simulink model "mars_rover_test_harness_chassis"  (R2025a)
settings: Solver=ode23t  StartTime=0.0  StopTime=30  FixedStep=1e-10  MaxStep=1e-1  RelTol=1e-3  AbsTol=1e-3  EnableMultiTasking=on
undefined symbols (not defined in the file): arm_q0, Control, L1, L2, L3, LS1, LS3, R1, R2, R3, Rover, RS1, RS3, X, Y, Z
libraries: sm_lib x119, nesl_utility x99, fl_lib x85, sdl_lib x20, ee_lib x10, mars_rover_lib x8, simulink x5, slpidlib x3, batteryecm_lib x2
(part 4 of 8)

== system mars_rover_test_harness_chassis/Rover/Chassis/Camera/rsm_base_1_RIGID ==
  ReferenceFrame : sm_lib/Frames and Transforms/Reference Frame
  Solid : sm_lib/Body Elements/File Solid  ExtGeomFileName=rover_chassis_sensor_base.stl  UnitType=Custom  ExtGeomFileUnits=cm  StepReaderType=HEX  ExportConvexHullGeometry=off  InertiaType=CalculateFromGeometry  BasedOnType=Density  Density=2000  DensityUnits=kg/m^3  Mass=202690.508551217  MassUnits=kg  CenterOfMass=[-2.09994238818055e-07 21.8231915316941 -2.20167989735098e-07]  CenterOfMassUnits=m  MomentsOfInertia=[2411866.97125594 5940029.20050206 6701187.74240286]  MomentsOfInertiaUnits=kg*m^2  ProductsOfInertia=[0.00792234309140369 -0.0164088810985133 -0.460936358460458]  ProductsOfInertiaUnits=kg*m^2  GraphicType=FromGeometry  MarkerShape=Sphere  MarkerSize=10  GraphicVisPropType=SimpleVisualProperties  GraphicDiffuseColor=[0.2 0.2 0.2]  GraphicOpacity=1  GraphicSpecularColor=[0.5 0.5 0.5 1.0]  GraphicAmbientColor=[0.15 0.15 0.15 1.0]  GraphicEmissiveColor=[0.0 0.0 0.0 1.0]  GraphicShininess=75  DoExposeReferenceFrame=on  SerializedFrames=<Frames/>
  Transform : sm_lib/Frames and Transforms/Rigid Transform  RotationMethod=ArbitraryAxis  FollAlignAxisA=+X  BaseAlignAxisA=+Y  FollAlignAxisB=+Y  BaseAlignAxisB=+Z  RotationStandardAxis=+Z  RotationAngle=2.0943951023932  RotationAngleUnits=rad  RotationArbitraryAxis=[0.577350269189626 0.577350269189626 0.577350269189626]  RotationSequenceAxes=FollowerAxes  RotationSequence=XYX  RotationSequenceAngles=[0 0 0]  RotationSequenceAnglesUnits=deg  RotationMatrix=[1 0 0; 0 1 0; 0 0 1]  Quaternion=[1 0 0 0]  TranslationMethod=Cartesian  TranslationCartesianOffset=[-40 220.000003786473 -2.05636384635e-06]  TranslationCartesianOffsetUnits=mm  TranslationStandardAxis=+Z  TranslationStandardOffset=0  TranslationStandardOffsetUnits=mm  TranslationROffset=0  TranslationROffsetUnits=m  TranslationThetaOffset=0  TranslationThetaOffsetUnits=deg  TranslationZOffset=0  TranslationZOffsetUnits=m
  F : PMIOPort  Side=Right
  F1 : PMIOPort  Port=2  Side=Left
  connections:
  Transform/LConn1 -- F1/RConn1 -- ReferenceFrame/RConn1 -- Solid/RConn1
  Transform/RConn1 -- F/RConn1

== system mars_rover_test_harness_chassis/Rover/Chassis/Camera/rsm_head_1_RIGID ==
  Reference Camera : sm_lib/Frames and Transforms/Reference Frame
  ReferenceFrame : sm_lib/Frames and Transforms/Reference Frame
  Rigid Transform : sm_lib/Frames and Transforms/Rigid Transform  RotationMethod=StandardAxis  FollAlignAxisA=+X  BaseAlignAxisA=+Y  FollAlignAxisB=+Y  BaseAlignAxisB=+Z  RotationStandardAxis=+X  RotationAngle=-90  RotationAngleUnits=deg  RotationArbitraryAxis=[0 0 1]  RotationSequenceAxes=FollowerAxes  RotationSequence=XYX  RotationSequenceAngles=[0 0 0]  RotationSequenceAnglesUnits=deg  RotationMatrix=[1 0 0; 0 1 0; 0 0 1]  Quaternion=[1 0 0 0]  TranslationMethod=Cartesian  TranslationCartesianOffset=[12 11 13]  TranslationCartesianOffsetUnits=cm  TranslationStandardAxis=+Z  TranslationStandardOffset=0  TranslationStandardOffsetUnits=cm  TranslationROffset=0  TranslationROffsetUnits=m  TranslationThetaOffset=0  TranslationThetaOffsetUnits=deg  TranslationZOffset=0  TranslationZOffsetUnits=m
  Solid : sm_lib/Body Elements/File Solid  ExtGeomFileName=rover_chassis_sensor_head.stl  UnitType=Custom  ExtGeomFileUnits=cm  StepReaderType=HEX  ExportConvexHullGeometry=off  InertiaType=CalculateFromGeometry  BasedOnType=Density  Density=2000  DensityUnits=kg/m^3  Mass=1  MassUnits=kg  CenterOfMass=[-0.00288550161429388 71.0000014663329 -4.54954138701768e-07]  CenterOfMassUnits=m  MomentsOfInertia=[1608495.92335293 6519098.97331966 6519098.97331985]  MomentsOfInertiaUnits=kg*m^2  ProductsOfInertia=[-6.49609544482223e-08 0.336731288221059 1.08955853960892]  ProductsOfInertiaUnits=kg*m^2  GraphicType=FromGeometry  MarkerShape=Sphere  MarkerSize=10  GraphicVisPropType=SimpleVisualProperties  GraphicDiffuseColor=[0.8 0.5 0.3]  GraphicOpacity=1  GraphicSpecularColor=[1 1 1 1.0]  GraphicAmbientColor=[0.15 0.15 0.15 0.8]  GraphicEmissiveColor=[0 0 0 1]  GraphicShininess=90  DoExposeReferenceFrame=on  SerializedFrames=<Frames/>
  Transform : sm_lib/Frames and Transforms/Rigid Transform  RotationMethod=ArbitraryAxis  FollAlignAxisA=+X  BaseAlignAxisA=+Y  FollAlignAxisB=+Y  BaseAlignAxisB=+Z  RotationStandardAxis=+Z  RotationAngle=2.0943951023932  RotationAngleUnits=rad  RotationArbitraryAxis=[0.577350269189626 0.577350269189626 0.577350269189626]  RotationSequenceAxes=FollowerAxes  RotationSequence=XYX  RotationSequenceAngles=[0 0 0]  RotationSequenceAnglesUnits=deg  RotationMatrix=[1 0 0; 0 1 0; 0 0 1]  Quaternion=[1 0 0 0]  TranslationMethod=Cartesian  TranslationCartesianOffset=[-40.5288600921631 710.000004438766 -7.70947271803379e-06]  TranslationCartesianOffsetUnits=mm  TranslationStandardAxis=+Z  TranslationStandardOffset=0  TranslationStandardOffsetUnits=mm  TranslationROffset=0  TranslationROffsetUnits=m  TranslationThetaOffset=0  TranslationThetaOffsetUnits=deg  TranslationZOffset=0  TranslationZOffsetUnits=m
  F : PMIOPort  Side=Left
  connections:
  ReferenceFrame/RConn1 -- Solid/RConn1 -- Transform/LConn1
  Transform/RConn1 -- F/RConn1 -- Rigid Transform/LConn1
  Rigid Transform/RConn1 -- Reference Camera/RConn1

== system mars_rover_test_harness_chassis/Rover/Chassis/Camera/rsm_lower_mast_2_RIGID ==
  ReferenceFrame : sm_lib/Frames and Transforms/Reference Frame
  Solid : sm_lib/Body Elements/File Solid  ExtGeomFileName=rover_chassis_sensor_mast_lower.stl  UnitType=Custom  ExtGeomFileUnits=cm  StepReaderType=HEX  ExportConvexHullGeometry=off  InertiaType=CalculateFromGeometry  BasedOnType=Density  Density=2000  DensityUnits=kg/m^3  Mass=403410.668072862  MassUnits=kg  CenterOfMass=[4.00000000041938 10.1119460218271 35.0000011171366]  CenterOfMassUnits=m  MomentsOfInertia=[4810006.95412572 3779509.77447628 5346172.06825756]  MomentsOfInertiaUnits=kg*m^2  ProductsOfInertia=[0.0256104910578052 9.59441184474277e-11 -0.00591852250388119]  ProductsOfInertiaUnits=kg*m^2  GraphicType=FromGeometry  MarkerShape=Sphere  MarkerSize=10  GraphicVisPropType=SimpleVisualProperties  GraphicDiffuseColor=[1 1 0.8]  GraphicOpacity=1  GraphicSpecularColor=[0.5 0.5 0.5 1.0]  GraphicAmbientColor=[0.15 0.15 0.15 1.0]  GraphicEmissiveColor=[0.0 0.0 0.0 1.0]  GraphicShininess=75  DoExposeReferenceFrame=on  SerializedFrames=<Frames/>
  Transform : sm_lib/Frames and Transforms/Rigid Transform  RotationMethod=ArbitraryAxis  FollAlignAxisA=+X  BaseAlignAxisA=+Y  FollAlignAxisB=+Y  BaseAlignAxisB=+Z  RotationStandardAxis=+Z  RotationAngle=2.0943951023932  RotationAngleUnits=rad  RotationArbitraryAxis=[-0.577350269189626 -0.577350269189626 -0.577350269189626]  RotationSequenceAxes=FollowerAxes  RotationSequence=XYX  RotationSequenceAngles=[0 0 0]  RotationSequenceAnglesUnits=deg  RotationMatrix=[1 0 0; 0 1 0; 0 0 1]  Quaternion=[1 0 0 0]  TranslationMethod=Cartesian  TranslationCartesianOffset=[40.0000013147577 450.900022888183 350.000005500325]  TranslationCartesianOffsetUnits=mm  TranslationStandardAxis=+Z  TranslationStandardOffset=0  TranslationStandardOffsetUnits=mm  TranslationROffset=0  TranslationROffsetUnits=m  TranslationThetaOffset=0  TranslationThetaOffsetUnits=deg  TranslationZOffset=0  TranslationZOffsetUnits=m
  Transform1 : sm_lib/Frames and Transforms/Rigid Transform  RotationMethod=ArbitraryAxis  FollAlignAxisA=+X  BaseAlignAxisA=+Y  FollAlignAxisB=+Y  BaseAlignAxisB=+Z  RotationStandardAxis=+Z  RotationAngle=2.0943951023932  RotationAngleUnits=rad  RotationArbitraryAxis=[0.577350269189626 0.577350269189626 0.577350269189626]  RotationSequenceAxes=FollowerAxes  RotationSequence=XYX  RotationSequenceAngles=[0 0 0]  RotationSequenceAnglesUnits=deg  RotationMatrix=[1 0 0; 0 1 0; 0 0 1]  Quaternion=[1 0 0 0]  TranslationMethod=Cartesian  TranslationCartesianOffset=[0 100.000002423247 350.000011189513]  TranslationCartesianOffsetUnits=mm  TranslationStandardAxis=+Z  TranslationStandardOffset=0  TranslationStandardOffsetUnits=mm  TranslationROffset=0  TranslationROffsetUnits=m  TranslationThetaOffset=0  TranslationThetaOffsetUnits=deg  TranslationZOffset=0  TranslationZOffsetUnits=m
  F1 : PMIOPort  Side=Left
  F : PMIOPort  Port=2  Side=Right
  connections:
  Transform/LConn1 -- Transform1/LConn1 -- ReferenceFrame/RConn1 -- Solid/RConn1
  Transform/RConn1 -- F/RConn1
  Transform1/RConn1 -- F1/RConn1

== system mars_rover_test_harness_chassis/Rover/Chassis/Camera/rsm_outer_ring_1_RIGID ==
  ReferenceFrame : sm_lib/Frames and Transforms/Reference Frame
  Rigid Transform : sm_lib/Frames and Transforms/Rigid Transform  RotationMethod=StandardAxis  FollAlignAxisA=+X  BaseAlignAxisA=+Y  FollAlignAxisB=+Y  BaseAlignAxisB=+Z  RotationStandardAxis=+Z  RotationAngle=20.0  RotationAngleUnits=deg  RotationArbitraryAxis=[0 0 1]  RotationSequenceAxes=FollowerAxes  RotationSequence=XYX  RotationSequenceAngles=[0 0 0]  RotationSequenceAnglesUnits=deg  RotationMatrix=[1 0 0; 0 1 0; 0 0 1]  Quaternion=[1 0 0 0]  TranslationMethod=None  TranslationCartesianOffset=[0 0 0]  TranslationCartesianOffsetUnits=m  TranslationStandardAxis=+Z  TranslationStandardOffset=0  TranslationStandardOffsetUnits=m  TranslationROffset=0  TranslationROffsetUnits=m  TranslationThetaOffset=0  TranslationThetaOffsetUnits=deg  TranslationZOffset=0  TranslationZOffsetUnits=m
  Solid : sm_lib/Body Elements/File Solid  ExtGeomFileName=rover_chassis_sensor_ring_outer.stl  UnitType=Custom  ExtGeomFileUnits=cm  StepReaderType=HEX  ExportConvexHullGeometry=off  InertiaType=CalculateFromGeometry  BasedOnType=Density  Density=2000  DensityUnits=kg/m^3  Mass=2000  MassUnits=kg  CenterOfMass=[3.99999986837507 43.0793255522792 35.0000003648552]  CenterOfMassUnits=m  MomentsOfInertia=[35996.0863503472 57529.9697773705 35996.0863503472]  MomentsOfInertiaUnits=kg*m^2  ProductsOfInertia=[0.000493832044278217 -4.64395705120422e-11 0.00068000513182705]  ProductsOfInertiaUnits=kg*m^2  GraphicType=FromGeometry  MarkerShape=Sphere  MarkerSize=10  GraphicVisPropType=SimpleVisualProperties  GraphicDiffuseColor=[0.2 0.2 0.2]  GraphicOpacity=1  GraphicSpecularColor=[0.5 0.5 0.5 1.0]  GraphicAmbientColor=[0.15 0.15 0.15 1.0]  GraphicEmissiveColor=[0.0 0.0 0.0 1.0]  GraphicShininess=75  DoExposeReferenceFrame=on  SerializedFrames=<Frames/>
  Transform : sm_lib/Frames and Transforms/Rigid Transform  RotationMethod=ArbitraryAxis  FollAlignAxisA=+X  BaseAlignAxisA=+Y  FollAlignAxisB=+Y  BaseAlignAxisB=+Z  RotationStandardAxis=+Z  RotationAngle=2.09439510239319  RotationAngleUnits=rad  RotationArbitraryAxis=[-0.577350269189626 -0.577350269189627 -0.577350269189625]  RotationSequenceAxes=FollowerAxes  RotationSequence=XYX  RotationSequenceAngles=[0 0 0]  RotationSequenceAnglesUnits=deg  RotationMatrix=[1 0 0; 0 1 0; 0 0 1]  Quaternion=[1 0 0 0]  TranslationMethod=Cartesian  TranslationCartesianOffset=[39.9999957537947 420.900022888184 350.000001520764]  TranslationCartesianOffsetUnits=mm  TranslationStandardAxis=+Z  TranslationStandardOffset=0  TranslationStandardOffsetUnits=mm  TranslationROffset=0  TranslationROffsetUnits=m  TranslationThetaOffset=0  TranslationThetaOffsetUnits=deg  TranslationZOffset=0  TranslationZOffsetUnits=m
  Transform1 : sm_lib/Frames and Transforms/Rigid Transform  RotationMethod=ArbitraryAxis  FollAlignAxisA=+X  BaseAlignAxisA=+Y  FollAlignAxisB=+Y  BaseAlignAxisB=+Z  RotationStandardAxis=+Z  RotationAngle=2.29441736937637  RotationAngleUnits=rad  RotationArbitraryAxis=[-0.450882585021863 -0.631151683244211 -0.631151683244211]  RotationSequenceAxes=FollowerAxes  RotationSequence=XYX  RotationSequenceAngles=[0 0 0]  RotationSequenceAnglesUnits=deg  RotationMatrix=[1 0 0; 0 1 0; 0 0 1]  Quaternion=[1 0 0 0]  TranslationMethod=Cartesian  TranslationCartesianOffset=[39.9999957537972 461.900007629394 350.000001520762]  TranslationCartesianOffsetUnits=mm  TranslationStandardAxis=+Z  TranslationStandardOffset=0  TranslationStandardOffsetUnits=mm  TranslationROffset=0  TranslationROffsetUnits=m  TranslationThetaOffset=0  TranslationThetaOffsetUnits=deg  TranslationZOffset=0  TranslationZOffsetUnits=m
  F1 : PMIOPort  Side=Left
  F : PMIOPort  Port=2  Side=Left
  connections:
  Transform/LConn1 -- Transform1/LConn1 -- ReferenceFrame/RConn1 -- Solid/RConn1
  Transform/RConn1 -- F/RConn1
  Rigid Transform/RConn1 -- F1/RConn1
  Rigid Transform/LConn1 -- Transform1/RConn1

== system mars_rover_test_harness_chassis/Rover/Chassis/Camera/rsm_upper_mast_1_RIGID ==
  ReferenceFrame : sm_lib/Frames and Transforms/Reference Frame
  Solid : sm_lib/Body Elements/File Solid  ExtGeomFileName=rover_chassis_sensor_mast_upper.stl  UnitType=Custom  ExtGeomFileUnits=cm  StepReaderType=HEX  ExportConvexHullGeometry=off  InertiaType=CalculateFromGeometry  BasedOnType=Density  Density=2000  DensityUnits=kg/m^3  Mass=382776.497765057  MassUnits=kg  CenterOfMass=[3.99998590581562 58.9787952931336 34.9999786232352]  CenterOfMassUnits=m  MomentsOfInertia=[3038949.11550358 3496444.12832479 3624138.33109519]  MomentsOfInertiaUnits=kg*m^2  ProductsOfInertia=[-149.383305940768 -0.0992863146641867 -86.2313374210248]  ProductsOfInertiaUnits=kg*m^2  GraphicType=FromGeometry  MarkerShape=Sphere  MarkerSize=10  GraphicVisPropType=SimpleVisualProperties  GraphicDiffuseColor=[1 1 0.8]  GraphicOpacity=1  GraphicSpecularColor=[0.5 0.5 0.5 1.0]  GraphicAmbientColor=[0.15 0.15 0.15 1.0]  GraphicEmissiveColor=[0.0 0.0 0.0 1.0]  GraphicShininess=75  DoExposeReferenceFrame=on  SerializedFrames=<Frames/>
  Transform : sm_lib/Frames and Transforms/Rigid Transform  RotationMethod=ArbitraryAxis  FollAlignAxisA=+X  BaseAlignAxisA=+Y  FollAlignAxisB=+Y  BaseAlignAxisB=+Z  RotationStandardAxis=+Z  RotationAngle=2.0943951023932  RotationAngleUnits=rad  RotationArbitraryAxis=[-0.577350269189626 -0.577350269189626 -0.577350269189626]  RotationSequenceAxes=FollowerAxes  RotationSequence=XYX  RotationSequenceAngles=[0 0 0]  RotationSequenceAnglesUnits=deg  RotationMatrix=[1 0 0; 0 1 0; 0 0 1]  Quaternion=[1 0 0 0]  TranslationMethod=Cartesian  TranslationCartesianOffset=[39.8936241533249 429.9 349.815749642353]  TranslationCartesianOffsetUnits=mm  TranslationStandardAxis=+Z  TranslationStandardOffset=0  TranslationStandardOffsetUnits=mm  TranslationROffset=0  TranslationROffsetUnits=m  TranslationThetaOffset=0  TranslationThetaOffsetUnits=deg  TranslationZOffset=0  TranslationZOffsetUnits=m
  Transform1 : sm_lib/Frames and Transforms/Rigid Transform  RotationMethod=ArbitraryAxis  FollAlignAxisA=+X  BaseAlignAxisA=+Y  FollAlignAxisB=+Y  BaseAlignAxisB=+Z  RotationStandardAxis=+Z  RotationAngle=2.0943951023932  RotationAngleUnits=rad  RotationArbitraryAxis=[0.577350269189626 0.577350269189626 0.577350269189626]  RotationSequenceAxes=FollowerAxes  RotationSequence=XYX  RotationSequenceAngles=[0 0 0]  RotationSequenceAnglesUnits=deg  RotationMatrix=[1 0 0; 0 1 0; 0 0 1]  Quaternion=[1 0 0 0]  TranslationMethod=Cartesian  TranslationCartesianOffset=[7.105427357601e-14 590.000009936775 350.000030393688]  TranslationCartesianOffsetUnits=mm  TranslationStandardAxis=+Z  TranslationStandardOffset=0  TranslationStandardOffsetUnits=mm  TranslationROffset=0  TranslationROffsetUnits=m  TranslationThetaOffset=0  TranslationThetaOffsetUnits=deg  TranslationZOffset=0  TranslationZOffsetUnits=m
  F : PMIOPort  Side=Left
  F1 : PMIOPort  Port=2  Side=Right
  connections:
  Transform/LConn1 -- Transform1/LConn1 -- ReferenceFrame/RConn1 -- Solid/RConn1
  Transform/RConn1 -- F/RConn1
  Transform1/RConn1 -- F1/RConn1

== system mars_rover_test_harness_chassis/Rover/Chassis/Powertrain/Electrical ==
  In Bus Element : Inport  PortName=Trq  Element=Steer
  In Bus Element1 : Inport  PortName=Trq  Element=Drive
  Drive : Subsystem  mask{trq_max=Rover.Powertrain.Drive.Motor.max_torque, power_max=Rover.Powertrain.Drive.Motor.max_power, trq_tc=Rover.Powertrain.Drive.Motor.tc_torque, eff_overall=Rover.Powertrain.Drive.Motor.efficiency, eff_spd=Rover.Powertrain.Drive.Motor.eff_meas_spd, eff_trq=Rover.Powertrain.Drive.Motor.eff_meas_trq, rotor_d=Rover.Powertrain.Drive.Motor.damping, drive_ratio=Rover.Powertrain.Drive.Motor.gear_ratio}
      mask prompts: trq_max "Max Torque (N*m)"; power_max "Max Power (W)"; trq_tc "Time Constant, Torque (s)"; eff_overall "Efficiency (%)"; eff_spd "Speed for Efficiency (rpm)"; eff_trq "Torque for Efficiency (N*m)"; rotor_d "Rotor Damping (N*m/(rad/s))"; drive_ratio "Drive Ratio"
      mask Display: image('mars_rover_terrain_motor_elec_drive.png');
  Mechanical Rotational Reference : fl_lib/Mechanical/Rotational Elements/Mechanical Rotational Reference
  Power : Subsystem
      mask Display: image('mars_rover_terrain_battery.png');
  Steer : Subsystem  mask{trq_max=Rover.Powertrain.Steer.Motor.max_torque, power_max=Rover.Powertrain.Steer.Motor.max_power, trq_tc=Rover.Powertrain.Steer.Motor.tc_torque, eff_overall=Rover.Powertrain.Steer.Motor.efficiency, eff_spd=Rover.Powertrain.Steer.Motor.eff_meas_spd, eff_trq=Rover.Powertrain.Steer.Motor.eff_meas_trq, rotor_d=Rover.Powertrain.Steer.Motor.damping, drive_ratio=Rover.Powertrain.Steer.Motor.gear_ratio}
      mask prompts: trq_max "Max Torque (N*m)"; power_max "Max Power (W)"; trq_tc "Time Constant, Torque (s)"; eff_overall "Efficiency (%)"; eff_spd "Speed for Efficiency (rpm)"; eff_trq "Torque for Efficiency (N*m)"; rotor_d "Rotor Damping (N*m/(rad/s))"; drive_ratio "Drive Ratio"
      mask Display: image('mars_rover_terrain_motor_elec_steer.png');
  S : PMIOPort  Side=Right
  Out Bus Element : Outport  PortName=m  Element=Drive
  Out Bus Element1 : Outport  PortName=m  Element=Steer
  Out Bus Element2 : Outport  PortName=m  Element=Battery
  wires:
  In Bus Element/1 -> Steer/1(Trq)
  In Bus Element1/1 -> Drive/1(Trq)
  Steer/1(m) -> Out Bus Element1/1
  Drive/1(m) -> Out Bus Element/1
  Power/1(m) -> Out Bus Element2/1
  connections:
  S/RConn1 -- Drive/RConn1 -- Steer/RConn1
  Power/RConn1 -- Drive/LConn1 -- Steer/LConn1
  Mechanical Rotational Reference/LConn1 -- Drive/RConn2 -- Steer/RConn2
  Power/RConn2 -- Drive/LConn2 -- Steer/LConn2

== system mars_rover_test_harness_chassis/Rover/Chassis/Powertrain/Ideal ==
  In Bus Element6 : Inport  PortName=Trq  Element=Steer
  In Bus Element : Inport  PortName=Trq  Element=Drive
  Calculate Power : Subsystem
  Drive : Subsystem  mask{drive_ratio=Rover.Powertrain.Drive.Motor.gear_ratio, motor_d=Rover.Powertrain.Drive.Motor.damping, motor_tc=Rover.Powertrain.Drive.Motor.tc_torque}
      mask prompts: drive_ratio "Drive Ratio"; motor_d "Motor Damping (N*m/(rad/s))"; motor_tc "Motor Time Constant"
      mask Display: image('mars_rover_terrain_motor_ideal_drive.png');
  Mechanical Rotational Reference : fl_lib/Mechanical/Rotational Elements/Mechanical Rotational Reference
  Power : Subsystem
      mask Display: image('mars_rover_terrain_battery.png');
  Steer : Subsystem  mask{drive_ratio=Rover.Powertrain.Drive.Motor.gear_ratio, motor_d=Rover.Powertrain.Steer.Motor.damping, motor_tc=Rover.Powertrain.Steer.Motor.tc_torque}
      mask prompts: drive_ratio "Gear Ratio"; motor_d "Motor Damping (N*m/(rad/s))"; motor_tc "Motor Time Constant"
      mask Display: image('mars_rover_terrain_motor_ideal_steer.png')
  S : PMIOPort  Side=Right
  Out Bus Element : Outport  PortName=m  Element=Steer
  Out Bus Element1 : Outport  PortName=m  Element=Drive
  Out Bus Element2 : Outport  PortName=m  Element=Battery
  wires:
  Steer/1(m) -> Out Bus Element/1, [S]
  In Bus Element6/1 -> Steer/1(Trq)
  Drive/1(m) -> [D], Out Bus Element1/1
  In Bus Element/1 -> Drive/1(Trq)
  [S] -> Calculate Power/1(S)
  [D] -> Calculate Power/2(D)
  Calculate Power/1(i) -> Power/1(i)
  Power/1(m) -> Out Bus Element2/1
  connections:
  Steer/RConn1 -- Drive/RConn1 -- S/RConn1
  Mechanical Rotational Reference/LConn1 -- Steer/LConn1 -- Drive/LConn1

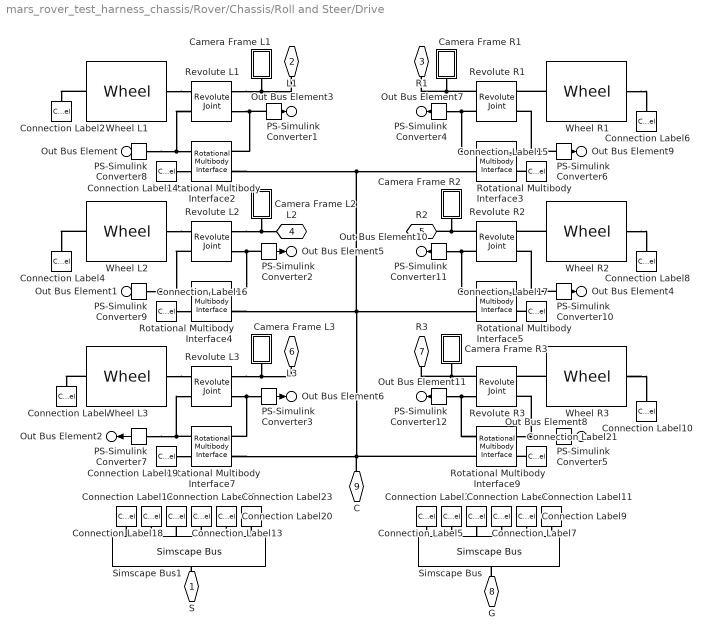
== system mars_rover_test_harness_chassis/Rover/Chassis/Roll and Steer/Drive ==
  Camera Frame L1 : Subsystem
  Camera Frame L2 : Subsystem
  Camera Frame L3 : Subsystem
  Camera Frame R1 : Subsystem
  Camera Frame R2 : Subsystem
  Camera Frame R3 : Subsystem
  Connection Label : ConnectionLabel  Label=GL3
  Connection Label1 : ConnectionLabel  Label=GL3
  Connection Label10 : ConnectionLabel  Label=GR3
  Connection Label11 : ConnectionLabel  Label=GR3
  Connection Label12 : ConnectionLabel  Label=L1
  Connection Label13 : ConnectionLabel  Label=R1
  Connection Label14 : ConnectionLabel  Label=L1
  Connection Label15 : ConnectionLabel  Label=R1
  Connection Label16 : ConnectionLabel  Label=L2
  Connection Label17 : ConnectionLabel  Label=R2
  Connection Label18 : ConnectionLabel  Label=L2
  Connection Label19 : ConnectionLabel  Label=L3
  Connection Label2 : ConnectionLabel  Label=GL1
  Connection Label20 : ConnectionLabel  Label=R2
  Connection Label21 : ConnectionLabel  Label=R3
  Connection Label22 : ConnectionLabel  Label=L3
  Connection Label23 : ConnectionLabel  Label=R3
  Connection Label3 : ConnectionLabel  Label=GL1
  Connection Label4 : ConnectionLabel  Label=GL2
  Connection Label5 : ConnectionLabel  Label=GL2
  Connection Label6 : ConnectionLabel  Label=GR1
  Connection Label7 : ConnectionLabel  Label=GR1
  Connection Label8 : ConnectionLabel  Label=GR2
  Connection Label9 : ConnectionLabel  Label=GR2
  PS-Simulink Converter{1..12} (12 alike) : nesl_utility/PS-Simulink Converter  PhysicalDomain=network_engine_domain  SubClassName=ps_output  LeftPortType=input  RightPortType=output  PseudoPeriodic=off  Frequencies=[]  VectorFormat=1-D array  Unit=inherit  AffineConversion=off
  Revolute L1 : sm_lib/Joints/Revolute Joint  JointMode=Normal  CompositeWrenchDir=FollowerOnBase  CompositeWrenchFrame=BaseFrame  SenseConstraintForce=off  SenseConstraintTorque=off  SenseTotalForce=off  SenseTotalTorque=off  PositionTargetSpecify=off  PositionTargetPriority=High  PositionTargetValue=0  PositionTargetValueUnits=deg  VelocityTargetSpecify=off  VelocityTargetPriority=High  VelocityTargetValue=0  VelocityTargetValueUnits=deg/s  EquilibriumPosition=0  EquilibriumPositionUnits=deg  SpringStiffness=0  SpringStiffnessUnits=N*m/deg  DampingCoefficient=Rover.Drive.D  DampingCoefficientUnits=N*m/(deg/s)  LowerLimitSpecify=off  LowerLimitBound=-90  LowerLimitBoundUnits=deg  LowerLimitStiffness=1e4  LowerLimitStiffnessUnits=N*m/deg  LowerLimitDamping=10  LowerLimitDampingUnits=N*m/(deg/s)  LowerLimitTransitionRegionWidth=0.1  LowerLimitTransitionRegionWidthUnits=deg  UpperLimitSpecify=off  UpperLimitBound=90  UpperLimitBoundUnits=deg  UpperLimitStiffness=1e4  UpperLimitStiffnessUnits=N*m/deg  UpperLimitDamping=10  UpperLimitDampingUnits=N*m/(deg/s)  UpperLimitTransitionRegionWidth=0.1  UpperLimitTransitionRegionWidthUnits=deg  TorqueActuationMode=InputTorque  MotionActuationMode=ComputedMotion  SensePosition=off  SenseVelocity=on  SenseAcceleration=off  SenseTorqueForce=off  SenseLowerLimitTorqueForce=off  SenseUpperLimitTorqueForce=off
  Revolute L2 : sm_lib/Joints/Revolute Joint  JointMode=Normal  CompositeWrenchDir=FollowerOnBase  CompositeWrenchFrame=BaseFrame  SenseConstraintForce=off  SenseConstraintTorque=off  SenseTotalForce=off  SenseTotalTorque=off  PositionTargetSpecify=off  PositionTargetPriority=High  PositionTargetValue=0  PositionTargetValueUnits=deg  VelocityTargetSpecify=off  VelocityTargetPriority=High  VelocityTargetValue=0  VelocityTargetValueUnits=deg/s  EquilibriumPosition=0  EquilibriumPositionUnits=deg  SpringStiffness=0  SpringStiffnessUnits=N*m/deg  DampingCoefficient=Rover.Drive.D  DampingCoefficientUnits=N*m/(deg/s)  LowerLimitSpecify=off  LowerLimitBound=-90  LowerLimitBoundUnits=deg  LowerLimitStiffness=1e4  LowerLimitStiffnessUnits=N*m/deg  LowerLimitDamping=10  LowerLimitDampingUnits=N*m/(deg/s)  LowerLimitTransitionRegionWidth=0.1  LowerLimitTransitionRegionWidthUnits=deg  UpperLimitSpecify=off  UpperLimitBound=90  UpperLimitBoundUnits=deg  UpperLimitStiffness=1e4  UpperLimitStiffnessUnits=N*m/deg  UpperLimitDamping=10  UpperLimitDampingUnits=N*m/(deg/s)  UpperLimitTransitionRegionWidth=0.1  UpperLimitTransitionRegionWidthUnits=deg  TorqueActuationMode=InputTorque  MotionActuationMode=ComputedMotion  SensePosition=off  SenseVelocity=on  SenseAcceleration=off  SenseTorqueForce=off  SenseLowerLimitTorqueForce=off  SenseUpperLimitTorqueForce=off
  Revolute L3 : sm_lib/Joints/Revolute Joint  JointMode=Normal  CompositeWrenchDir=FollowerOnBase  CompositeWrenchFrame=BaseFrame  SenseConstraintForce=off  SenseConstraintTorque=off  SenseTotalForce=off  SenseTotalTorque=off  PositionTargetSpecify=off  PositionTargetPriority=High  PositionTargetValue=0  PositionTargetValueUnits=deg  VelocityTargetSpecify=off  VelocityTargetPriority=High  VelocityTargetValue=0  VelocityTargetValueUnits=deg/s  EquilibriumPosition=0  EquilibriumPositionUnits=deg  SpringStiffness=0  SpringStiffnessUnits=N*m/deg  DampingCoefficient=Rover.Drive.D  DampingCoefficientUnits=N*m/(deg/s)  LowerLimitSpecify=off  LowerLimitBound=-90  LowerLimitBoundUnits=deg  LowerLimitStiffness=1e4  LowerLimitStiffnessUnits=N*m/deg  LowerLimitDamping=10  LowerLimitDampingUnits=N*m/(deg/s)  LowerLimitTransitionRegionWidth=0.1  LowerLimitTransitionRegionWidthUnits=deg  UpperLimitSpecify=off  UpperLimitBound=90  UpperLimitBoundUnits=deg  UpperLimitStiffness=1e4  UpperLimitStiffnessUnits=N*m/deg  UpperLimitDamping=10  UpperLimitDampingUnits=N*m/(deg/s)  UpperLimitTransitionRegionWidth=0.1  UpperLimitTransitionRegionWidthUnits=deg  TorqueActuationMode=InputTorque  MotionActuationMode=ComputedMotion  SensePosition=off  SenseVelocity=on  SenseAcceleration=off  SenseTorqueForce=off  SenseLowerLimitTorqueForce=off  SenseUpperLimitTorqueForce=off
  Revolute R1 : sm_lib/Joints/Revolute Joint  JointMode=Normal  CompositeWrenchDir=FollowerOnBase  CompositeWrenchFrame=BaseFrame  SenseConstraintForce=off  SenseConstraintTorque=off  SenseTotalForce=off  SenseTotalTorque=off  PositionTargetSpecify=off  PositionTargetPriority=High  PositionTargetValue=0  PositionTargetValueUnits=deg  VelocityTargetSpecify=off  VelocityTargetPriority=High  VelocityTargetValue=0  VelocityTargetValueUnits=deg/s  EquilibriumPosition=0  EquilibriumPositionUnits=deg  SpringStiffness=0  SpringStiffnessUnits=N*m/deg  DampingCoefficient=Rover.Drive.D  DampingCoefficientUnits=N*m/(deg/s)  LowerLimitSpecify=off  LowerLimitBound=-90  LowerLimitBoundUnits=deg  LowerLimitStiffness=1e4  LowerLimitStiffnessUnits=N*m/deg  LowerLimitDamping=10  LowerLimitDampingUnits=N*m/(deg/s)  LowerLimitTransitionRegionWidth=0.1  LowerLimitTransitionRegionWidthUnits=deg  UpperLimitSpecify=off  UpperLimitBound=90  UpperLimitBoundUnits=deg  UpperLimitStiffness=1e4  UpperLimitStiffnessUnits=N*m/deg  UpperLimitDamping=10  UpperLimitDampingUnits=N*m/(deg/s)  UpperLimitTransitionRegionWidth=0.1  UpperLimitTransitionRegionWidthUnits=deg  TorqueActuationMode=InputTorque  MotionActuationMode=ComputedMotion  SensePosition=off  SenseVelocity=on  SenseAcceleration=off  SenseTorqueForce=off  SenseLowerLimitTorqueForce=off  SenseUpperLimitTorqueForce=off
  Revolute R2 : sm_lib/Joints/Revolute Joint  JointMode=Normal  CompositeWrenchDir=FollowerOnBase  CompositeWrenchFrame=BaseFrame  SenseConstraintForce=off  SenseConstraintTorque=off  SenseTotalForce=off  SenseTotalTorque=off  PositionTargetSpecify=off  PositionTargetPriority=High  PositionTargetValue=0  PositionTargetValueUnits=deg  VelocityTargetSpecify=off  VelocityTargetPriority=High  VelocityTargetValue=0  VelocityTargetValueUnits=deg/s  EquilibriumPosition=0  EquilibriumPositionUnits=deg  SpringStiffness=0  SpringStiffnessUnits=N*m/deg  DampingCoefficient=Rover.Drive.D  DampingCoefficientUnits=N*m/(deg/s)  LowerLimitSpecify=off  LowerLimitBound=-90  LowerLimitBoundUnits=deg  LowerLimitStiffness=1e4  LowerLimitStiffnessUnits=N*m/deg  LowerLimitDamping=10  LowerLimitDampingUnits=N*m/(deg/s)  LowerLimitTransitionRegionWidth=0.1  LowerLimitTransitionRegionWidthUnits=deg  UpperLimitSpecify=off  UpperLimitBound=90  UpperLimitBoundUnits=deg  UpperLimitStiffness=1e4  UpperLimitStiffnessUnits=N*m/deg  UpperLimitDamping=10  UpperLimitDampingUnits=N*m/(deg/s)  UpperLimitTransitionRegionWidth=0.1  UpperLimitTransitionRegionWidthUnits=deg  TorqueActuationMode=InputTorque  MotionActuationMode=ComputedMotion  SensePosition=off  SenseVelocity=on  SenseAcceleration=off  SenseTorqueForce=off  SenseLowerLimitTorqueForce=off  SenseUpperLimitTorqueForce=off
  Revolute R3 : sm_lib/Joints/Revolute Joint  JointMode=Normal  CompositeWrenchDir=FollowerOnBase  CompositeWrenchFrame=BaseFrame  SenseConstraintForce=off  SenseConstraintTorque=off  SenseTotalForce=off  SenseTotalTorque=off  PositionTargetSpecify=off  PositionTargetPriority=High  PositionTargetValue=0  PositionTargetValueUnits=deg  VelocityTargetSpecify=off  VelocityTargetPriority=High  VelocityTargetValue=0  VelocityTargetValueUnits=deg/s  EquilibriumPosition=0  EquilibriumPositionUnits=deg  SpringStiffness=0  SpringStiffnessUnits=N*m/deg  DampingCoefficient=Rover.Drive.D  DampingCoefficientUnits=N*m/(deg/s)  LowerLimitSpecify=off  LowerLimitBound=-90  LowerLimitBoundUnits=deg  LowerLimitStiffness=1e4  LowerLimitStiffnessUnits=N*m/deg  LowerLimitDamping=10  LowerLimitDampingUnits=N*m/(deg/s)  LowerLimitTransitionRegionWidth=0.1  LowerLimitTransitionRegionWidthUnits=deg  UpperLimitSpecify=off  UpperLimitBound=90  UpperLimitBoundUnits=deg  UpperLimitStiffness=1e4  UpperLimitStiffnessUnits=N*m/deg  UpperLimitDamping=10  UpperLimitDampingUnits=N*m/(deg/s)  UpperLimitTransitionRegionWidth=0.1  UpperLimitTransitionRegionWidthUnits=deg  TorqueActuationMode=InputTorque  MotionActuationMode=ComputedMotion  SensePosition=off  SenseVelocity=on  SenseAcceleration=off  SenseTorqueForce=off  SenseLowerLimitTorqueForce=off  SenseUpperLimitTorqueForce=off
  Rotational Multibody Interface{2..5,7,9} (6 alike) : fl_lib/Mechanical/Multibody Interfaces/Rotational Multibody Interface
  Simscape Bus : SimscapeBus  HierarchyStrings=L1;L2;L3;R1;R2;R3
  Simscape Bus1 : SimscapeBus  HierarchyStrings=L1;L2;L3;R1;R2;R3
  Wheel L1 : mars_rover_lib/Wheel  popup_leftRight=Left  pt_cld_loc=Rover.Wheel.wheel_point_cloud  pt_cld_rad=Rover.Wheel.point_cloud_vis.rad  pt_cld_clr=Rover.Wheel.point_cloud_vis.clr  pt_cld_opc=Rover.Wheel.point_cloud_vis.opc
  Wheel L2 : mars_rover_lib/Wheel  popup_leftRight=Left  pt_cld_loc=Rover.Wheel.wheel_point_cloud  pt_cld_rad=Rover.Wheel.point_cloud_vis.rad  pt_cld_clr=Rover.Wheel.point_cloud_vis.clr  pt_cld_opc=Rover.Wheel.point_cloud_vis.opc
  Wheel L3 : mars_rover_lib/Wheel  popup_leftRight=Left  pt_cld_loc=Rover.Wheel.wheel_point_cloud  pt_cld_rad=Rover.Wheel.point_cloud_vis.rad  pt_cld_clr=Rover.Wheel.point_cloud_vis.clr  pt_cld_opc=Rover.Wheel.point_cloud_vis.opc
  Wheel R1 : mars_rover_lib/Wheel  popup_leftRight=Right  pt_cld_loc=Rover.Wheel.wheel_point_cloud  pt_cld_rad=Rover.Wheel.point_cloud_vis.rad  pt_cld_clr=Rover.Wheel.point_cloud_vis.clr  pt_cld_opc=Rover.Wheel.point_cloud_vis.opc
  Wheel R2 : mars_rover_lib/Wheel  popup_leftRight=Right  pt_cld_loc=Rover.Wheel.wheel_point_cloud  pt_cld_rad=Rover.Wheel.point_cloud_vis.rad  pt_cld_clr=Rover.Wheel.point_cloud_vis.clr  pt_cld_opc=Rover.Wheel.point_cloud_vis.opc
  Wheel R3 : mars_rover_lib/Wheel  popup_leftRight=Right  pt_cld_loc=Rover.Wheel.wheel_point_cloud  pt_cld_rad=Rover.Wheel.point_cloud_vis.rad  pt_cld_clr=Rover.Wheel.point_cloud_vis.clr  pt_cld_opc=Rover.Wheel.point_cloud_vis.opc
  S : PMIOPort  Side=Left
  L1 : PMIOPort  Port=2  Side=Left
  R1 : PMIOPort  Port=3  Side=Right
  L2 : PMIOPort  Port=4  Side=Left
  R2 : PMIOPort  Port=5  Side=Right
  L3 : PMIOPort  Port=6  Side=Left
  R3 : PMIOPort  Port=7  Side=Right
  G : PMIOPort  Port=8  Side=Right
  C : PMIOPort  Port=9  Side=Left
  Out Bus Element : Outport  PortName=m  Element=w.L1
  Out Bus Element1 : Outport  PortName=m  Element=w.L2
  Out Bus Element2 : Outport  PortName=m  Element=w.L3
  Out Bus Element9 : Outport  PortName=m  Element=w.R1
  Out Bus Element4 : Outport  PortName=m  Element=w.R2
  Out Bus Element8 : Outport  PortName=m  Element=w.R3
  Out Bus Element3 : Outport  PortName=m  Element=trq.L1
  Out Bus Element5 : Outport  PortName=m  Element=trq.L2
  Out Bus Element6 : Outport  PortName=m  Element=trq.L3
  Out Bus Element7 : Outport  PortName=m  Element=trq.R1
  Out Bus Element10 : Outport  PortName=m  Element=trq.R2
  Out Bus Element11 : Outport  PortName=m  Element=trq.R3
  wires:
  PS-Simulink Converter7/1 -> Out Bus Element2/1
  PS-Simulink Converter5/1 -> Out Bus Element8/1
  PS-Simulink Converter9/1 -> Out Bus Element1/1
  PS-Simulink Converter6/1 -> Out Bus Element9/1
  PS-Simulink Converter8/1 -> Out Bus Element/1
  PS-Simulink Converter10/1 -> Out Bus Element4/1
  PS-Simulink Converter1/1 -> Out Bus Element3/1
  PS-Simulink Converter2/1 -> Out Bus Element5/1
  PS-Simulink Converter3/1 -> Out Bus Element6/1
  PS-Simulink Converter4/1 -> Out Bus Element7/1
  PS-Simulink Converter11/1 -> Out Bus Element10/1
  PS-Simulink Converter12/1 -> Out Bus Element11/1
  connections:
  Revolute L1/LConn2 -- PS-Simulink Converter1/LConn1 -- Rotational Multibody Interface2/LConn1
  Connection Label17/LConn1 -- Rotational Multibody Interface5/RConn2
  Wheel L2/RConn1 -- Revolute L2/RConn1
  Wheel L1/RConn1 -- Revolute L1/RConn1
  Connection Label3/LConn1 -- Simscape Bus/LConn1
  Rotational Multibody Interface7/RConn1 -- Revolute L3/RConn2 -- PS-Simulink Converter7/LConn1
  Connection Label9/LConn1 -- Simscape Bus/LConn5
  Wheel R3/LConn1 -- Connection Label10/LConn1
  Wheel R3/RConn1 -- Revolute R3/RConn1
  Revolute L2/RConn2 -- PS-Simulink Converter9/LConn1 -- Rotational Multibody Interface4/RConn1
  Rotational Multibody Interface3/RConn1 -- Revolute R1/RConn2 -- PS-Simulink Converter6/LConn1
  Rotational Multibody Interface4/LConn2 -- Rotational Multibody Interface7/LConn2 -- C/RConn1 -- Rotational Multibody Interface9/LConn2 -- Rotational Multibody Interface2/LConn2 -- Rotational Multibody Interface3/LConn2 -- Rotational Multibody Interface5/LConn2
  Connection Label1/LConn1 -- Simscape Bus/LConn3
  Revolute L1/RConn2 -- PS-Simulink Converter8/LConn1 -- Rotational Multibody Interface2/RConn1
  Connection Label5/LConn1 -- Simscape Bus/LConn2
  Wheel R1/LConn1 -- Connection Label6/LConn1
  Wheel R2/LConn1 -- Connection Label8/LConn1
  Revolute R1/LConn1 -- R1/RConn1 -- Camera Frame R1/LConn1
  Wheel L1/LConn1 -- Connection Label2/LConn1
  Rotational Multibody Interface9/RConn1 -- Revolute R3/RConn2 -- PS-Simulink Converter5/LConn1
  G/RConn1 -- Simscape Bus/RConn1
  Connection Label14/LConn1 -- Rotational Multibody Interface2/RConn2
  Wheel R2/RConn1 -- Revolute R2/RConn1
  Connection Label7/LConn1 -- Simscape Bus/LConn4
  Revolute L2/LConn1 -- Camera Frame L2/LConn1 -- L2/RConn1
  Wheel R1/RConn1 -- Revolute R1/RConn1
  Wheel L2/LConn1 -- Connection Label4/LConn1
  Connection Label15/LConn1 -- Rotational Multibody Interface3/RConn2
  Revolute R1/LConn2 -- Rotational Multibody Interface3/LConn1 -- PS-Simulink Converter4/LConn1
  Connection Label21/LConn1 -- Rotational Multibody Interface9/RConn2
  Wheel L3/RConn1 -- Revolute L3/RConn1
  Revolute L3/LConn2 -- PS-Simulink Converter3/LConn1 -- Rotational Multibody Interface7/LConn1
  Connection Label19/LConn1 -- Rotational Multibody Interface7/RConn2
  Rotational Multibody Interface5/RConn1 -- Revolute R2/RConn2 -- PS-Simulink Converter10/LConn1
  Revolute R2/LConn1 -- Camera Frame R2/LConn1 -- R2/RConn1
  Revolute L3/LConn1 -- Camera Frame L3/LConn1 -- L3/RConn1
  Rotational Multibody Interface9/LConn1 -- PS-Simulink Converter12/LConn1 -- Revolute R3/LConn2
  Revolute L1/LConn1 -- L1/RConn1 -- Camera Frame L1/LConn1
  Connection Label11/LConn1 -- Simscape Bus/LConn6
  Revolute L2/LConn2 -- PS-Simulink Converter2/LConn1 -- Rotational Multibody Interface4/LConn1
  Connection Label16/LConn1 -- Rotational Multibody Interface4/RConn2
  Wheel L3/LConn1 -- Connection Label/LConn1
  Revolute R2/LConn2 -- PS-Simulink Converter11/LConn1 -- Rotational Multibody Interface5/LConn1
  Revolute R3/LConn1 -- R3/RConn1 -- Camera Frame R3/LConn1
  Simscape Bus1/LConn1 -- Connection Label12/LConn1
  Simscape Bus1/LConn2 -- Connection Label18/LConn1
  Simscape Bus1/LConn3 -- Connection Label22/LConn1
  Simscape Bus1/LConn4 -- Connection Label13/LConn1
  Simscape Bus1/LConn5 -- Connection Label20/LConn1
  Simscape Bus1/LConn6 -- Connection Label23/LConn1
  S/RConn1 -- Simscape Bus1/RConn1

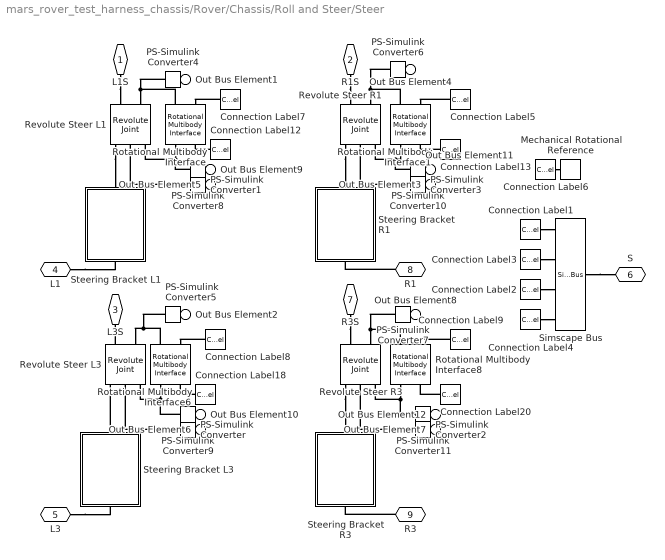
== system mars_rover_test_harness_chassis/Rover/Chassis/Roll and Steer/Steer ==
  Connection Label1 : ConnectionLabel  Label=LS1
  Connection Label12 : ConnectionLabel  Label=LS1
  Connection Label13 : ConnectionLabel  Label=RS1
  Connection Label18 : ConnectionLabel  Label=LS3
  Connection Label2 : ConnectionLabel  Label=RS1
  Connection Label20 : ConnectionLabel  Label=RS3
  Connection Label3 : ConnectionLabel  Label=LS3
  Connection Label4 : ConnectionLabel  Label=RS3
  Connection Label{5..9} (5 alike) : ConnectionLabel  Label=C
  Mechanical Rotational Reference : fl_lib/Mechanical/Rotational Elements/Mechanical Rotational Reference
  PS-Simulink Converter{,1..3} (4 alike) : nesl_utility/PS-Simulink Converter  PhysicalDomain=network_engine_domain  SubClassName=ps_output  LeftPortType=input  RightPortType=output  PseudoPeriodic=off  Frequencies=[]  VectorFormat=1-D array  Unit=deg  AffineConversion=off
  PS-Simulink Converter{4..11} (8 alike) : nesl_utility/PS-Simulink Converter  PhysicalDomain=network_engine_domain  SubClassName=ps_output  LeftPortType=input  RightPortType=output  PseudoPeriodic=off  Frequencies=[]  VectorFormat=1-D array  Unit=inherit  AffineConversion=off
  Revolute Steer L1 : sm_lib/Joints/Revolute Joint  JointMode=Normal  CompositeWrenchDir=FollowerOnBase  CompositeWrenchFrame=BaseFrame  SenseConstraintForce=off  SenseConstraintTorque=off  SenseTotalForce=off  SenseTotalTorque=off  PositionTargetSpecify=on  PositionTargetPriority=High  PositionTargetValue=0  PositionTargetValueUnits=deg  VelocityTargetSpecify=off  VelocityTargetPriority=High  VelocityTargetValue=0  VelocityTargetValueUnits=deg/s  EquilibriumPosition=0  EquilibriumPositionUnits=deg  SpringStiffness=0  SpringStiffnessUnits=N*m/deg  DampingCoefficient=Rover.Steer.D  DampingCoefficientUnits=N*m/(deg/s)  LowerLimitSpecify=off  LowerLimitBound=-90  LowerLimitBoundUnits=deg  LowerLimitStiffness=1e4  LowerLimitStiffnessUnits=N*m/deg  LowerLimitDamping=10  LowerLimitDampingUnits=N*m/(deg/s)  LowerLimitTransitionRegionWidth=0.1  LowerLimitTransitionRegionWidthUnits=deg  UpperLimitSpecify=off  UpperLimitBound=90  UpperLimitBoundUnits=deg  UpperLimitStiffness=1e4  UpperLimitStiffnessUnits=N*m/deg  UpperLimitDamping=10  UpperLimitDampingUnits=N*m/(deg/s)  UpperLimitTransitionRegionWidth=0.1  UpperLimitTransitionRegionWidthUnits=deg  TorqueActuationMode=InputTorque  MotionActuationMode=ComputedMotion  SensePosition=on  SenseVelocity=on  SenseAcceleration=off  SenseTorqueForce=off  SenseLowerLimitTorqueForce=off  SenseUpperLimitTorqueForce=off
  Revolute Steer L3 : sm_lib/Joints/Revolute Joint  JointMode=Normal  CompositeWrenchDir=FollowerOnBase  CompositeWrenchFrame=BaseFrame  SenseConstraintForce=off  SenseConstraintTorque=off  SenseTotalForce=off  SenseTotalTorque=off  PositionTargetSpecify=on  PositionTargetPriority=High  PositionTargetValue=0  PositionTargetValueUnits=deg  VelocityTargetSpecify=off  VelocityTargetPriority=High  VelocityTargetValue=0  VelocityTargetValueUnits=deg/s  EquilibriumPosition=0  EquilibriumPositionUnits=deg  SpringStiffness=0  SpringStiffnessUnits=N*m/deg  DampingCoefficient=Rover.Steer.D  DampingCoefficientUnits=N*m/(deg/s)  LowerLimitSpecify=off  LowerLimitBound=-90  LowerLimitBoundUnits=deg  LowerLimitStiffness=1e4  LowerLimitStiffnessUnits=N*m/deg  LowerLimitDamping=10  LowerLimitDampingUnits=N*m/(deg/s)  LowerLimitTransitionRegionWidth=0.1  LowerLimitTransitionRegionWidthUnits=deg  UpperLimitSpecify=off  UpperLimitBound=90  UpperLimitBoundUnits=deg  UpperLimitStiffness=1e4  UpperLimitStiffnessUnits=N*m/deg  UpperLimitDamping=10  UpperLimitDampingUnits=N*m/(deg/s)  UpperLimitTransitionRegionWidth=0.1  UpperLimitTransitionRegionWidthUnits=deg  TorqueActuationMode=InputTorque  MotionActuationMode=ComputedMotion  SensePosition=on  SenseVelocity=on  SenseAcceleration=off  SenseTorqueForce=off  SenseLowerLimitTorqueForce=off  SenseUpperLimitTorqueForce=off
  Revolute Steer R1 : sm_lib/Joints/Revolute Joint  JointMode=Normal  CompositeWrenchDir=FollowerOnBase  CompositeWrenchFrame=BaseFrame  SenseConstraintForce=off  SenseConstraintTorque=off  SenseTotalForce=off  SenseTotalTorque=off  PositionTargetSpecify=on  PositionTargetPriority=High  PositionTargetValue=0  PositionTargetValueUnits=deg  VelocityTargetSpecify=off  VelocityTargetPriority=High  VelocityTargetValue=0  VelocityTargetValueUnits=deg/s  EquilibriumPosition=0  EquilibriumPositionUnits=deg  SpringStiffness=0  SpringStiffnessUnits=N*m/deg  DampingCoefficient=Rover.Steer.D  DampingCoefficientUnits=N*m/(deg/s)  LowerLimitSpecify=off  LowerLimitBound=-90  LowerLimitBoundUnits=deg  LowerLimitStiffness=1e4  LowerLimitStiffnessUnits=N*m/deg  LowerLimitDamping=10  LowerLimitDampingUnits=N*m/(deg/s)  LowerLimitTransitionRegionWidth=0.1  LowerLimitTransitionRegionWidthUnits=deg  UpperLimitSpecify=off  UpperLimitBound=90  UpperLimitBoundUnits=deg  UpperLimitStiffness=1e4  UpperLimitStiffnessUnits=N*m/deg  UpperLimitDamping=10  UpperLimitDampingUnits=N*m/(deg/s)  UpperLimitTransitionRegionWidth=0.1  UpperLimitTransitionRegionWidthUnits=deg  TorqueActuationMode=InputTorque  MotionActuationMode=ComputedMotion  SensePosition=on  SenseVelocity=on  SenseAcceleration=off  SenseTorqueForce=off  SenseLowerLimitTorqueForce=off  SenseUpperLimitTorqueForce=off
  Revolute Steer R3 : sm_lib/Joints/Revolute Joint  JointMode=Normal  CompositeWrenchDir=FollowerOnBase  CompositeWrenchFrame=BaseFrame  SenseConstraintForce=off  SenseConstraintTorque=off  SenseTotalForce=off  SenseTotalTorque=off  PositionTargetSpecify=on  PositionTargetPriority=High  PositionTargetValue=0  PositionTargetValueUnits=deg  VelocityTargetSpecify=off  VelocityTargetPriority=High  VelocityTargetValue=0  VelocityTargetValueUnits=deg/s  EquilibriumPosition=0  EquilibriumPositionUnits=deg  SpringStiffness=0  SpringStiffnessUnits=N*m/deg  DampingCoefficient=Rover.Steer.D  DampingCoefficientUnits=N*m/(deg/s)  LowerLimitSpecify=off  LowerLimitBound=-90  LowerLimitBoundUnits=deg  LowerLimitStiffness=1e4  LowerLimitStiffnessUnits=N*m/deg  LowerLimitDamping=10  LowerLimitDampingUnits=N*m/(deg/s)  LowerLimitTransitionRegionWidth=0.1  LowerLimitTransitionRegionWidthUnits=deg  UpperLimitSpecify=off  UpperLimitBound=90  UpperLimitBoundUnits=deg  UpperLimitStiffness=1e4  UpperLimitStiffnessUnits=N*m/deg  UpperLimitDamping=10  UpperLimitDampingUnits=N*m/(deg/s)  UpperLimitTransitionRegionWidth=0.1  UpperLimitTransitionRegionWidthUnits=deg  TorqueActuationMode=InputTorque  MotionActuationMode=ComputedMotion  SensePosition=on  SenseVelocity=on  SenseAcceleration=off  SenseTorqueForce=off  SenseLowerLimitTorqueForce=off  SenseUpperLimitTorqueForce=off
  Rotational Multibody Interface{,1,6,8} (4 alike) : fl_lib/Mechanical/Multibody Interfaces/Rotational Multibody Interface
  Simscape Bus : SimscapeBus  HierarchyStrings=LS1;LS3;RS1;RS3
  Steering Bracket L1 : Subsystem
      mask Display: image('mars_rover_terrain_chassis_steerbracketl.png');
  Steering Bracket L3 : Subsystem
      mask Display: image('mars_rover_terrain_chassis_steerbracketl.png');
  Steering Bracket R1 : Subsystem
      mask Display: image('mars_rover_terrain_chassis_steerbracketr.png');
  Steering Bracket R3 : Subsystem
      mask Display: image('mars_rover_terrain_chassis_steerbracketr.png');
  L1S : PMIOPort  Side=Left
  R1S : PMIOPort  Port=2  Side=Right
  L3S : PMIOPort  Port=3  Side=Left
  L1 : PMIOPort  Port=4  Side=Left
  L3 : PMIOPort  Port=5  Side=Left
  S : PMIOPort  Port=6  Side=Left
  R3S : PMIOPort  Port=7  Side=Right
  R1 : PMIOPort  Port=8  Side=Right
  R3 : PMIOPort  Port=9  Side=Right
  Out Bus Element5 : Outport  PortName=m  Element=q.L1
  Out Bus Element6 : Outport  PortName=m  Element=q.L3
  Out Bus Element3 : Outport  PortName=m  Element=q.R1
  Out Bus Element7 : Outport  PortName=m  Element=q.R3
  Out Bus Element2 : Outport  PortName=m  Element=trq.L3
  Out Bus Element1 : Outport  PortName=m  Element=trq.L1
  Out Bus Element4 : Outport  PortName=m  Element=trq.R1
  Out Bus Element8 : Outport  PortName=m  Element=trq.R3
  Out Bus Element9 : Outport  PortName=m  Element=w.L1
  Out Bus Element10 : Outport  PortName=m  Element=w.L2
  Out Bus Element11 : Outport  PortName=m  Element=w.R1
  Out Bus Element12 : Outport  PortName=m  Element=w.R3
  wires:
  PS-Simulink Converter3/1 -> Out Bus Element3/1
  PS-Simulink Converter1/1 -> Out Bus Element5/1
  PS-Simulink Converter/1 -> Out Bus Element6/1
  PS-Simulink Converter2/1 -> Out Bus Element7/1
  PS-Simulink Converter4/1 -> Out Bus Element1/1
  PS-Simulink Converter5/1 -> Out Bus Element2/1
  PS-Simulink Converter6/1 -> Out Bus Element4/1
  PS-Simulink Converter7/1 -> Out Bus Element8/1
  PS-Simulink Converter8/1 -> Out Bus Element9/1
  PS-Simulink Converter9/1 -> Out Bus Element10/1
  PS-Simulink Converter10/1 -> Out Bus Element11/1
  PS-Simulink Converter11/1 -> Out Bus Element12/1
  connections:
  Rotational Multibody Interface1/RConn1 -- Revolute Steer R1/RConn3 -- PS-Simulink Converter10/LConn1
  Rotational Multibody Interface1/LConn1 -- PS-Simulink Converter6/LConn1 -- Revolute Steer R1/LConn2
  Rotational Multibody Interface/LConn1 -- PS-Simulink Converter4/LConn1 -- Revolute Steer L1/LConn2
  Connection Label8/LConn1 -- Rotational Multibody Interface6/LConn2
  Revolute Steer R1/RConn1 -- Steering Bracket R1/RConn1
  Connection Label18/LConn1 -- Rotational Multibody Interface6/RConn2
  Connection Label7/LConn1 -- Rotational Multibody Interface/LConn2
  Connection Label9/LConn1 -- Rotational Multibody Interface8/LConn2
  Steering Bracket L3/LConn1 -- Revolute Steer L3/RConn1
  Revolute Steer R3/RConn1 -- Steering Bracket R3/RConn1
  Connection Label5/LConn1 -- Rotational Multibody Interface1/LConn2
  L1S/RConn1 -- Revolute Steer L1/LConn1
  Rotational Multibody Interface/RConn1 -- Revolute Steer L1/RConn3 -- PS-Simulink Converter8/LConn1
  Rotational Multibody Interface8/RConn1 -- Revolute Steer R3/RConn3 -- PS-Simulink Converter11/LConn1
  Revolute Steer L1/RConn1 -- Steering Bracket L1/LConn1
  Connection Label13/LConn1 -- Rotational Multibody Interface1/RConn2
  R3S/RConn1 -- Revolute Steer R3/LConn1
  Rotational Multibody Interface6/LConn1 -- PS-Simulink Converter5/LConn1 -- Revolute Steer L3/LConn2
  Revolute Steer L3/LConn1 -- L3S/RConn1
  R1/RConn1 -- Steering Bracket R1/LConn1
  Connection Label20/LConn1 -- Rotational Multibody Interface8/RConn2
  R3/RConn1 -- Steering Bracket R3/LConn1
  Rotational Multibody Interface8/LConn1 -- PS-Simulink Converter7/LConn1 -- Revolute Steer R3/LConn2
  R1S/RConn1 -- Revolute Steer R1/LConn1
  Rotational Multibody Interface6/RConn1 -- Revolute Steer L3/RConn3 -- PS-Simulink Converter9/LConn1
  Connection Label12/LConn1 -- Rotational Multibody Interface/RConn2
  L1/RConn1 -- Steering Bracket L1/RConn1
  L3/RConn1 -- Steering Bracket L3/RConn1
  Connection Label1/LConn1 -- Simscape Bus/LConn1
  Connection Label3/LConn1 -- Simscape Bus/LConn2
  Connection Label2/LConn1 -- Simscape Bus/LConn3
  Connection Label4/LConn1 -- Simscape Bus/LConn4
  Simscape Bus/RConn1 -- S/RConn1
  PS-Simulink Converter1/LConn1 -- Revolute Steer L1/RConn2
  PS-Simulink Converter3/LConn1 -- Revolute Steer R1/RConn2
  PS-Simulink Converter/LConn1 -- Revolute Steer L3/RConn2
  PS-Simulink Converter2/LConn1 -- Revolute Steer R3/RConn2
  Connection Label6/LConn1 -- Mechanical Rotational Reference/LConn1
